simulink model "rms_variant"  (R2025a)
settings: Solver=FixedStepDiscrete  StartTime=0.0  StopTime=stopTime  FixedStep=MST  MaxStep=1  RelTol=1e-3  EnableMultiTasking=on
undefined symbols (not defined in the file): lvdtOffsetDig, maxRatio, maxStroke, samplePeriod, samplesPerCycle
libraries: dspstat3 x2, simulink x2
settings Model: Creator=mbrun  LastModifiedBy=mbrun
settings DataIOCC: SaveOutput=off  SignalLogging=off  DSMLogging=off  StreamToWks=off  SaveTime=off  ReturnWorkspaceOutputs=off
settings OptimizationCC: DefaultParameterBehavior=Inlined  EnhancedBackFolding=on  PassReuseOutputArgsAs=Individual arguments  ZeroExternalMemoryAtStartup=off  ZeroInternalMemoryAtStartup=off  MaxStackSize=64  OptimizeBlockOrder=speed  DifferentSizesBufferReuse=on  OptimizationCustomize=off  EfficientTunableParamExpr=on
settings DebuggingCC: ParameterTunabilityLossMsg=error  SFUnexpectedBacktrackingDiag=warning  SFNoUnconditionalDefaultTransitionDiag=warning
settings HardwareCC: ProdBitPerPointer=32.0  ProdBitPerSizeT=32.0  ProdBitPerPtrDiffT=32.0  ProdLargestAtomicInteger=Long  ProdLargestAtomicFloat=Double  ProdWordSize=32.0  ProdHWDeviceType=NXP->Cortex-M0/M0+
settings SFSimCC: MATLABDynamicMemAlloc=off
settings RTWCC: SystemTargetFile=ert.tlc  GenCodeOnly=on  PackageGeneratedCodeAndArtifacts=on  TemplateMakefile=ert_default_tmf  Toolchain=GNU Tools for ARM Embedded Processors  BuildConfiguration=Debug  Description=Embedded Coder
settings CodeAppCC: ForceParamTrailComments=on  IgnoreCustomStorageClasses=off  OperatorAnnotations=on  SimulinkDataObjDesc=on  SFDataObjDesc=on  InsertBlockDesc=on  EnableCustomComments=on
settings ERTTargetCC: ExtModeTransport=0.0  ExtModeStaticAlloc=off  ExtModeMexFile=ext_comm  ExtModeIntrfLevel=Level1  ERTCustomFileTemplate=example_file_process.tlc

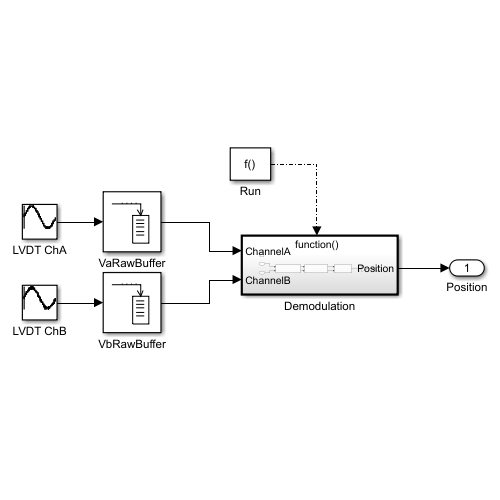
[thumbnail: Simulink's stored preview of the top-level diagram]
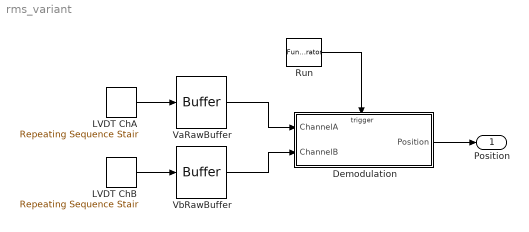
== system rms_variant ==
  Demodulation : Subsystem  TreatAsAtomicUnit=on
  LVDT ChA : simulink/Sources/Repeating Sequence Stair  OutValues=adcSignalA  tsamp=samplePeriod  OutMin=[]  OutMax=[]  OutDataTypeStr=uint16  OutputDataTypeScalingMode=uint16  OutDataType=fixdt(0,8)  ConRadixGroup=Best Precision: Vector-wise  OutScaling=2^-12
  LVDT ChB : simulink/Sources/Repeating Sequence Stair  OutValues=adcSignalB  tsamp=samplePeriod  OutMin=[]  OutMax=[]  OutDataTypeStr=uint16  OutputDataTypeScalingMode=uint16  OutDataType=fixdt(0,8)  ConRadixGroup=Best Precision: Vector-wise  OutScaling=2^-12
  Run : FunctionCallGenerator  SampleTime=samplePeriod*samplesPerCycle
  VaRawBuffer : Buffer  N=samplesPerCycle
  VbRawBuffer : Buffer  N=samplesPerCycle
  Position : Outport  OutDataTypeStr=double
  wires:
  Demodulation/1(Position) -> Position/1
  VaRawBuffer/1 -> Demodulation/1(ChannelA)
  Run/1 -> Demodulation/Trigger
  VbRawBuffer/1 -> Demodulation/2(ChannelB)
  LVDT ChA/1 -> VaRawBuffer/1
  LVDT ChB/1 -> VbRawBuffer/1

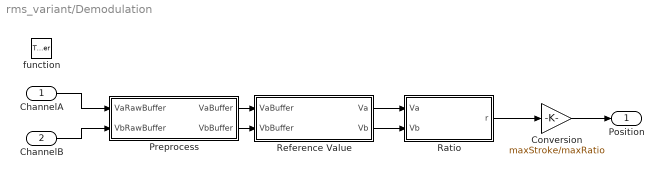
== system rms_variant/Demodulation ==
  ChannelA : Inport  OutDataTypeStr=uint16
  ChannelB : Inport  Port=2  OutDataTypeStr=uint16
  function : TriggerPort  TriggerType=function-call  VariantControl=(inherit)
  Conversion : Gain  Gain=maxStroke/maxRatio  OutDataTypeStr=double
  Preprocess : Subsystem
  Ratio : Subsystem
  Reference Value : Subsystem
  Position : Outport  OutDataTypeStr=double
  wires:
  Preprocess/2(VbBuffer) -> Reference Value/2(VbBuffer)
  Ratio/1(r) -> Conversion/1
  ChannelB/1 -> Preprocess/2(VbRawBuffer)
  Reference Value/1(Va) -> Ratio/1(Va)
  Preprocess/1(VaBuffer) -> Reference Value/1(VaBuffer)
  Conversion/1 -> Position/1
  Reference Value/2(Vb) -> Ratio/2(Vb)
  ChannelA/1 -> Preprocess/1(VaRawBuffer)

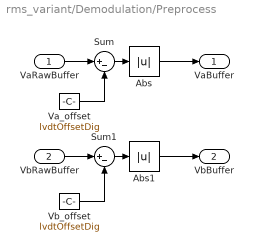
== system rms_variant/Demodulation/Preprocess ==
  VaRawBuffer : Inport  OutDataTypeStr=uint16
  VbRawBuffer : Inport  Port=2  OutDataTypeStr=uint16
  Abs : Abs  OutDataTypeStr=double  SaturateOnIntegerOverflow=off
  Abs1 : Abs  OutDataTypeStr=double  SaturateOnIntegerOverflow=off
  Sum : Sum  Inputs=|+-  OutDataTypeStr=double
  Sum1 : Sum  Inputs=|+-  OutDataTypeStr=double
  Va_offset : Constant  Value=lvdtOffsetDig
  Vb_offset : Constant  Value=lvdtOffsetDig
  VaBuffer : Outport  OutDataTypeStr=double
  VbBuffer : Outport  Port=2  OutDataTypeStr=double
  wires:
  Abs/1 -> VaBuffer/1
  Abs1/1 -> VbBuffer/1
  Vb_offset/1 -> Sum1/2
  VaRawBuffer/1 -> Sum/1
  Sum/1 -> Abs/1
  Va_offset/1 -> Sum/2
  Sum1/1 -> Abs1/1
  VbRawBuffer/1 -> Sum1/1

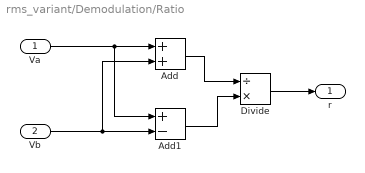
== system rms_variant/Demodulation/Ratio ==
  Va : Inport  OutDataTypeStr=double
  Vb : Inport  Port=2  OutDataTypeStr=double
  Add : Sum
  Add1 : Sum  Inputs=+-
  Divide : Product  Inputs=/*
  r : Outport  OutDataTypeStr=double
  wires:
  Vb/1 -> Add/2, Add1/2
  Add1/1 -> Divide/2
  Add/1 -> Divide/1
  Va/1 -> Add1/1, Add/1
  Divide/1 -> r/1

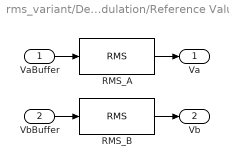
== system rms_variant/Demodulation/Reference Value ==
  VaBuffer : Inport  OutDataTypeStr=double
  VbBuffer : Inport  Port=2  OutDataTypeStr=double
  RMS_A : dspstat3/RMS  run=off  directionMode=Each column  dimension=1  InputProcessing=Columns as channels (frame based)  reset_popup=None
  RMS_B : dspstat3/RMS  run=off  directionMode=Each column  dimension=1  InputProcessing=Columns as channels (frame based)  reset_popup=None
  Va : Outport  OutDataTypeStr=double
  Vb : Outport  Port=2  OutDataTypeStr=double
  wires:
  VaBuffer/1 -> RMS_A/1
  RMS_A/1 -> Va/1
  VbBuffer/1 -> RMS_B/1
  RMS_B/1 -> Vb/1
